simulink model "Ch15Ex3"  (Simulink 4.00)
settings: Solver=ode45  StartTime=0.0  StopTime=7  RelTol=1e-3

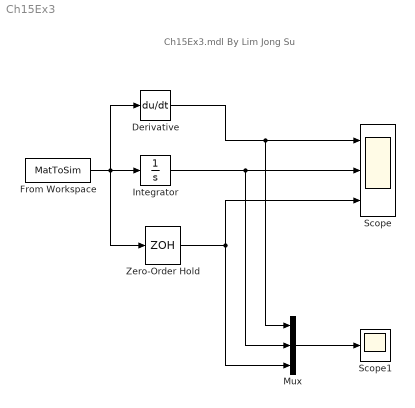
== system Ch15Ex3 ==
  note: Ch15Ex3.mdl
      | By Lim Jong Su
  Derivative : Derivative
  From Workspace : FromWorkspace  VariableName=MatToSim  SampleTime=0.1  OutputAfterFinalValue=Extrapolation
  Integrator : Integrator  ExternalReset=none  InitialConditionSource=internal  InitialCondition=0  LimitOutput=off  UpperSaturationLimit=inf  LowerSaturationLimit=-inf  ShowSaturationPort=off  ShowStatePort=off  AbsoluteTolerance=auto
  Mux : Mux  Inputs=3
  Scope : Scope  NumInputPorts=3
      settings: TimeRange=auto  YMin=-5~-5~-5  YMax=5~5~5  SaveToWorkspace=off  SaveName=ScopeData  LimitDataPoints=on  MaxDataPoints=5000
  Scope1 : Scope
      settings: TimeRange=auto  YMin=-5  YMax=5  SaveToWorkspace=off  LimitDataPoints=on  MaxDataPoints=5000
  Zero-Order Hold : ZeroOrderHold  SampleTime=0.5
  wires:
  From Workspace/1 -> Integrator/1, Derivative/1, Zero-Order Hold/1
  Integrator/1 -> Scope/2, Mux/2
  Derivative/1 -> Scope/1, Mux/1
  Zero-Order Hold/1 -> Scope/3, Mux/3
  Mux/1 -> Scope1/1
